simulink model "Tractor_HIT_Discrete"  (R2024a)
settings: Solver=ode1  StartTime=0.0  StopTime=60  FixedStep=0.001  RelTol=1e-3
values from neighbouring files (symbols this model uses):
  ANRtarget = 1.05    [Engine1204.sldd]    (also in Engine1204_init_r1.m; Engine2004.sldd; Engine2004_init.m; Engine3204.sldd)
  BackPrs = 3.0 4.2 5.5 7.0 8.5 10.0 11.5 12.5    [Engine1204.sldd]    (also in Engine1204_init_r1.m = [3.0, 4.2, 5.5, 7.0, 8.5, 10.0, 11.5, 12.5]; Engine2004.sldd = 3.0 4.2 5.5 7.0 8.5 10.0 11.5 12.5 13.5 14.5 15.0 15.5 16.0 ; Engine2004_init.m = [3.0,4.2,5.5,7.0,8.5,10.0,11.5,12.5,13.5,14.5,15.0,15.5,16.0; Engine3204.sldd = 3.0 4.5 6.0 7.5 9.0 10.5 12.0 13.0 13.8 14.4 14.8 15.2 15.6 )
  BackPrs_x = 50.0 100.0 150.0 200.0 250.0 300.0 350.0 400.0    [Engine1204.sldd]    (also in Engine1204_init_r1.m = [50:50:400]; Engine2004.sldd = 50.0 100.0 150.0 200.0 250.0 300.0 350.0 400.0 450.0 500.0 5; Engine2004_init.m = [50:50:800]; Engine3204.sldd = 100.0 200.0 300.0 400.0 500.0 600.0 700.0 800.0 900.0 1000.0)
  Bf = 0.38    [Engine1204.sldd]    (also in Engine2004.sldd; Engine3204.sldd)
  Br = 0.47    [Engine1204.sldd]    (also in Engine2004.sldd; Engine3204.sldd)
  BSFC = 320.0 285.0 275.0 280.0 290.0 300.0 310.0 260.0 225.0 215.0 220.0 228.0 240.0 250.0 235.0 208.0 202.0 205.0 212.0 222.0 232.0 230.0 205.0 200.0 204.0 210.0 220.0 230.0 232.0 207.0 203.0 206.0 213.0 224.0 235.0    [Engine1204.sldd]    (also in Engine1204_init_r1.m = [320,285,275,280,290,300,310; Engine2004.sldd = 315.0 280.0 270.0 275.0 285.0 295.0 305.0 255.0 220.0 210.0 ; Engine2004_init.m = [315,280,270,275,285,295,305; Engine3204.sldd = 310.0 275.0 265.0 270.0 280.0 290.0 300.0 250.0 215.0 205.0 )
  BSFC_x = 700.0 1200.0 1400.0 1600.0 1800.0 2000.0 2200.0    [Engine1204.sldd]    (also in Engine1204_init_r1.m = [700,1200,1400,1600,1800,2000,2200]; Engine2004.sldd = 800.0 1200.0 1400.0 1600.0 1800.0 2000.0 2200.0; Engine2004_init.m = [800,1200,1400,1600,1800,2000,2200]; Engine3204.sldd = 800.0 1000.0 1200.0 1400.0 1600.0 1800.0 2100.0)
  BSFC_y = 12.0 24.0 36.0 48.0 54.0    [Engine1204.sldd]    (also in Engine1204_init_r1.m = [12,24,36,48,54]; Engine2004.sldd = 20.0 40.0 60.0 80.0 100.0; Engine2004_init.m = [20,40,60,80,100]; Engine3204.sldd = 30.0 60.0 90.0 120.0 150.0)
  CO = 2.4 1.7 1.5 1.6 1.8 2.1 2.7 1.1 0.72 0.65 0.68 0.78 0.92 1.3 0.7 0.55 0.5 0.53 0.6 0.72 0.95 1.2 0.9 0.85 0.88 0.96 1.1 1.45 3.2 2.3 2.1 2.25 2.5 2.85 3.8    [Engine1204.sldd]    (also in Engine1204_init_r1.m = [; Engine2004.sldd = 2.3 1.63 1.44 1.54 1.73 2.02 2.56 1.05 0.68 0.61 0.64 0.74 0; Engine2004_init.m = [; Engine3204.sldd = 2.2 1.56 1.38 1.48 1.66 1.94 2.46 1.0 0.65 0.58 0.61 0.7 0.8)
  CO_x = 700.0 1200.0 1400.0 1600.0 1800.0 2000.0 2200.0    [Engine1204.sldd]    (also in Engine1204_init_r1.m = [700,1200,1400,1600,1800,2000,2200]; Engine2004.sldd = 800.0 1200.0 1400.0 1600.0 1800.0 2000.0 2200.0; Engine2004_init.m = [800,1200,1400,1600,1800,2000,2200]; Engine3204.sldd = 800.0 1000.0 1200.0 1400.0 1600.0 1800.0 2100.0)
  CO_y = 12.0 24.0 36.0 48.0 54.0    [Engine1204.sldd]    (also in Engine1204_init_r1.m = [12,24,36,48,54]; Engine2004.sldd = 20.0 40.0 60.0 80.0 100.0; Engine2004_init.m = [20,40,60,80,100]; Engine3204.sldd = 30.0 60.0 90.0 120.0 150.0)
  Df = 1.4    [Engine1204.sldd]    (also in Engine2004.sldd; Engine3204.sldd)
  dfmax = 0.1    [Engine1204.sldd]    (also in Engine2004.sldd; Engine3204.sldd)
  dfmin = 0.035    [Engine1204.sldd]    (also in Engine2004.sldd; Engine3204.sldd)
  DOCdPrs = 0.2 0.5 0.8 1.1 1.2    [Engine1204.sldd]    (also in Engine1204_init_r1.m = [0.2  0.5  0.8  1.1  1.2]; Engine2004.sldd = 0.25 0.55 0.85 1.15 1.3; Engine2004_init.m = [0.25,0.55,0.85,1.15,1.30]; Engine3204.sldd = 0.25 0.55 0.85 1.15 1.3 1.45)
  DOCdPrs_x = 50.0 150.0 250.0 350.0 400.0    [Engine1204.sldd]    (also in Engine1204_init_r1.m = [50  150  250  350  400]; Engine2004.sldd = 100.0 250.0 400.0 600.0 800.0; Engine2004_init.m = [100 250 400 600 800]; Engine3204.sldd = 100.0 250.0 400.0 600.0 800.0 1200.0)
  DPFdPrs = 0.3 0.5 0.7 0.9 0.6 1.0 1.4 1.8 0.9 1.5 2.1 2.6 1.2 2.0 2.7 2.8    [Engine1204.sldd]    (also in Engine1204_init_r1.m = [0.3  0.5  0.7  0.9; Engine2004.sldd = 0.35 0.6 0.85 1.1 0.7 1.15 1.6 2.0 1.05 1.7 2.3 2.5 1.4 2.2 ; Engine2004_init.m = [0.35,0.60,0.85,1.10; Engine3204.sldd = 0.35 0.7 1.05 1.4 1.7 2.0 2.2 2.4 2.55 2.65 2.7 2.75 0.6 1.1)
  DPFdPrs_x = 100.0 200.0 300.0 400.0    [Engine1204.sldd]    (also in Engine1204_init_r1.m = [100: 100 : 400]; Engine2004.sldd = 100.0 300.0 500.0 700.0; Engine2004_init.m = [100:200:700]; Engine3204.sldd = 100.0 200.0 300.0 400.0 500.0 600.0 700.0 800.0 900.0 1000.0)
  DPFdPrs_y = 0.0 6.0 12.0 20.0    [Engine1204.sldd]    (also in Engine1204_init_r1.m = [0 6 12 20 ]; Engine2004.sldd = 0.0 8.0 16.0 24.0; Engine2004_init.m = [0 8 16 24]; Engine3204.sldd = 0.0 10.0 20.0 30.0)
  DPFSootBurn = 0.0 0.0 0.0 0.0 0.0 0.2 0.4 0.6 0.8 1.0 1.2 2.4 3.6 4.8 6.0 6.0 12.0 18.0 24.0 30.0 12.0 24.0 36.0 48.0 60.0 20.0 40.0 60.0 80.0 100.0 22.0 44.0 66.0 88.0 110.0    [Engine1204.sldd]    (also in Engine1204_init_r1.m = [0,0,0,0,0; Engine2004.sldd = 0.0 0.0 0.0 0.0 0.0 0.5 1.0 1.5 2.0 2.5 3.0 6.0 9.0 12.0 15.; Engine2004_init.m = [0,0,0,0,0; Engine3204.sldd = 0.0 0.0 0.0 0.0 0.0 0.5 1.0 1.5 2.0 2.5 3.0 6.0 9.0 12.0 15.)
  DPFSootBurn_x = 100.0 200.0 300.0 400.0 500.0    [Engine1204.sldd]    (also in Engine1204_init_r1.m = [100,200,300,400,500]; Engine2004.sldd = 200.0 300.0 400.0 500.0 650.0; Engine2004_init.m = [200,300,400,500,650]; Engine3204.sldd = 200.0 300.0 400.0 500.0 650.0)
  DPFSootBurn_y = 400.0 450.0 500.0 550.0 600.0 650.0 680.0    [Engine1204.sldd]    (also in Engine1204_init_r1.m = [400,450,500,550,600,650,680]; Engine2004.sldd; Engine2004_init.m = [400,450,500,550,600,650,680]; Engine3204.sldd)
  Dr = 1.8    [Engine1204.sldd]    (also in Engine2004.sldd; Engine3204.sldd)
  drmax = 0.12    [Engine1204.sldd]    (also in Engine2004.sldd; Engine3204.sldd)
  drmin = 0.04    [Engine1204.sldd]    (also in Engine2004.sldd; Engine3204.sldd)
  EGRKi = 0.03    [Engine1204.sldd]    (also in Engine1204_init_r1.m; Engine2004.sldd; Engine2004_init.m; Engine3204.sldd)
  EGRKp = 3.5999999999999996    [Engine1204.sldd]    (also in Engine1204_init_r1.m = 3.6; Engine2004.sldd; Engine2004_init.m = 3.6; Engine3204.sldd)
  EGRMax = 1.0    [Engine1204.sldd]    (also in Engine1204_init_r1.m = 1; Engine2004.sldd; Engine2004_init.m = 1; Engine3204.sldd)
  EGRMin = 0.0    [Engine1204.sldd]    (also in Engine1204_init_r1.m = 0; Engine2004.sldd; Engine2004_init.m = 0; Engine3204.sldd)
  EGRRatio = 0.0 0.0 0.0 0.0 0.0 0.0 0.0 0.0 0.04 0.03 0.03 0.02 0.02 0.01 0.0 0.08 0.07 0.06 0.05 0.04 0.03 0.0 0.13 0.12 0.11 0.1 0.09 0.08 0.0 0.18 0.17 0.16 0.15 0.14 0.13 0.0 0.22 0.21 0.2 0.19 0.18 0.17    [Engine1204.sldd]    (also in Engine1204_init_r1.m = [; Engine2004.sldd; Engine2004_init.m = [; Engine3204.sldd)
  EGRRatio_x = 700.0 1200.0 1400.0 1600.0 1800.0 2000.0 2200.0    [Engine1204.sldd]    (also in Engine1204_init_r1.m = [700,1200,1400,1600,1800,2000,2200]; Engine2004.sldd = 800.0 1200.0 1400.0 1600.0 1800.0 2000.0 2200.0; Engine2004_init.m = [800,1200,1400,1600,1800,2000,2200]; Engine3204.sldd = 800.0 1000.0 1200.0 1400.0 1600.0 1800.0 2100.0)
  EGRRatio_y = 0.0 20.0 40.0 60.0 80.0 100.0    [Engine1204.sldd]    (also in Engine1204_init_r1.m = [0,20,40,60,80,100]; Engine2004.sldd; Engine2004_init.m = [0,20,40,60,80,100]; Engine3204.sldd)
  EGRTgt = 0.25 0.22 0.2 0.18 0.16 0.12 0.1 0.2 0.18 0.15 0.14 0.12 0.1 0.08 0.12 0.13 0.1 0.09 0.08 0.06 0.04 0.08 0.09 0.07 0.06 0.05 0.03 0.02 0.05 0.06 0.04 0.03 0.02 0.01 0.0    [Engine1204.sldd]    (also in Engine1204_init_r1.m = [0.25,0.22,0.20,0.18,0.16,0.12,0.10; Engine2004.sldd = 0.24 0.21 0.19 0.17 0.15 0.11 0.09 0.19 0.17 0.14 0.13 0.11 ; Engine2004_init.m = [0.24,0.21,0.19,0.17,0.15,0.11,0.09; Engine3204.sldd = 0.23 0.2 0.18 0.16 0.14 0.1 0.08 0.18 0.16 0.13 0.12 0.1 0.0)
  EGRTgt_x = 700.0 1200.0 1400.0 1600.0 1800.0 2000.0 2200.0    [Engine1204.sldd]    (also in Engine1204_init_r1.m = [700,1200,1400,1600,1800,2000,2200]; Engine2004.sldd = 800.0 1200.0 1400.0 1600.0 1800.0 2000.0 2200.0; Engine2004_init.m = [800,1200,1400,1600,1800,2000,2200]; Engine3204.sldd = 800.0 1000.0 1200.0 1400.0 1600.0 1800.0 2100.0)
  EGRTgt_y = 12.0 24.0 36.0 48.0 54.0    [Engine1204.sldd]    (also in Engine1204_init_r1.m = [12,24,36,48,54]; Engine2004.sldd = 20.0 40.0 60.0 80.0 100.0; Engine2004_init.m = [20,40,60,80,100]; Engine3204.sldd = 30.0 60.0 90.0 120.0 150.0)
  EGT = 197.0 257.0 287.0 297.0 287.0 267.0 247.0 267.0 357.0 397.0 407.0 392.0 367.0 347.0 337.0 437.0 472.0 482.0 462.0 437.0 407.0 367.0 477.0 502.0 512.0 492.0 467.0 437.0 377.0 487.0 510.0 520.0 500.0 477.0 447.0    [Engine1204.sldd]    (also in Engine1204_init_r1.m = [470,530,560,570,560,540,520; Engine2004.sldd = 187.0 247.0 277.0 287.0 277.0 257.0 237.0 257.0 347.0 387.0 ; Engine2004_init.m = [460,520,550,560,550,530,510; Engine3204.sldd = 307.0 327.0 338.0 327.0 307.0 277.0 237.0 322.0 337.0 332.0 )
  EGT_x = 700.0 1200.0 1400.0 1600.0 1800.0 2000.0 2200.0    [Engine1204.sldd]    (also in Engine1204_init_r1.m = [700,1200,1400,1600,1800,2000,2200]; Engine2004.sldd = 800.0 1200.0 1400.0 1600.0 1800.0 2000.0 2200.0; Engine2004_init.m = [800,1200,1400,1600,1800,2000,2200]; Engine3204.sldd = 800.0 1000.0 1200.0 1400.0 1600.0 1800.0 2100.0)
  EGT_y = 12.0 24.0 36.0 48.0 54.0    [Engine1204.sldd]    (also in Engine1204_init_r1.m = [12,24,36,48,54]; Engine2004.sldd = 20.0 40.0 60.0 80.0 100.0; Engine2004_init.m = [20,40,60,80,100]; Engine3204.sldd = 30.0 60.0 90.0 120.0 150.0)
  EngCsup = 0.35594 0.35501499999999997 0.353535 0.35242500000000004 0.351685 0.35150000000000003 0.35187 0.352795 0.35446 0.356865    [Engine1204.sldd]    (also in Engine2004.sldd; Engine3204.sldd)
  EngineSpdTgt = 700.0 850.0 1000.0 1150.0 1300.0 1450.0 1600.0 1750.0 1900.0 2050.0 2200.0    [Engine1204.sldd]    (also in Engine1204_init_r1.m = [700:150:2200]; Engine2004.sldd; Engine2004_init.m = [700:150:2200]; Engine3204.sldd = 800.0 930.0 1060.0 1190.0 1320.0 1450.0 1580.0 1710.0 1840.0)
  EngineSpdTgt_x = 0.0 10.0 20.0 30.0 40.0 50.0 60.0 70.0 80.0 90.0 100.0    [Engine1204.sldd]    (also in Engine1204_init_r1.m = [0:10:100]; Engine2004.sldd; Engine2004_init.m = [0:10:100]; Engine3204.sldd)
  EngineTrq = 70.0 110.0 130.0 125.0 115.0 100.0 85.0 180.0 280.0 320.0 310.0 285.0 250.0 220.0 260.0 370.0 410.0 395.0 365.0 320.0 280.0 300.0 420.0 450.0 435.0 400.0 350.0 300.0 310.0 435.0 460.0 445.0 410.0 355.0 305.0    [Engine1204.sldd]    (also in Engine1204_init_r1.m = [70,110,130,125,115,100,85; Engine2004.sldd = 130.0 200.0 240.0 230.0 210.0 180.0 150.0 320.0 480.0 550.0 ; Engine2004_init.m = [130,200,240,230,210,180,150; Engine3204.sldd = 210.0 320.0 380.0 360.0 330.0 290.0 240.0 510.0 760.0 870.0 )
  EngineTrq_x = 700.0 1200.0 1400.0 1600.0 1800.0 2000.0 2200.0    [Engine1204.sldd]    (also in Engine1204_init_r1.m = [700,1200,1400,1600,1800,2000,2200]; Engine2004.sldd = 800.0 1200.0 1400.0 1600.0 1800.0 2000.0 2200.0; Engine2004_init.m = [800,1200,1400,1600,1800,2000,2200]; Engine3204.sldd = 800.0 1000.0 1200.0 1400.0 1600.0 1800.0 2100.0)
  EngineTrq_y = 12.0 24.0 36.0 48.0 54.0    [Engine1204.sldd]    (also in Engine1204_init_r1.m = [12,24,36,48,54]; Engine2004.sldd = 20.0 40.0 60.0 80.0 100.0; Engine2004_init.m = [20,40,60,80,100]; Engine3204.sldd = 30.0 60.0 90.0 120.0 150.0)
  EngSpd = 800.0 1000.0 1200.0 1400.0 1600.0 1800.0 2000.0 2200.0 2400.0 2600.0    [Engine1204.sldd]    (also in Engine2004.sldd; Engine3204.sldd)
  EngTrq = 667.0 700.0 768.0 830.0 885.0 860.0 789.0 690.0 542.0 352.0    [Engine1204.sldd]    (also in Engine2004.sldd; Engine3204.sldd)
  etaCO = 0.0 0.0 0.0 0.0 0.6 0.45 0.3 0.15 0.92 0.85 0.75 0.6 0.98 0.95 0.9 0.82 0.99 0.97 0.94 0.88    [Engine1204.sldd]    (also in Engine1204_init_r1.m = [0.00	0.00	0.00	0.00; Engine2004.sldd; Engine2004_init.m = [0.00	0.00	0.00	0.00; Engine3204.sldd)
  etaCO_x = 10000.0 25000.0 40000.0 60000.0    [Engine1204.sldd]    (also in Engine1204_init_r1.m = [10000  25000  40000  60000]; Engine2004.sldd; Engine2004_init.m = [10000 25000 40000 60000]; Engine3204.sldd)
  etaCO_y = 120.0 200.0 280.0 360.0 450.0    [Engine1204.sldd]    (also in Engine1204_init_r1.m = [120, 200, 280, 360, 450]; Engine2004.sldd; Engine2004_init.m = [120,200,280,360,450]; Engine3204.sldd)
  etaHC = 0.0 0.0 0.0 0.0 0.5 0.35 0.2 0.1 0.88 0.8 0.68 0.5 0.96 0.92 0.86 0.75 0.98 0.95 0.91 0.83    [Engine1204.sldd]    (also in Engine1204_init_r1.m = [0.00	0.00	0.00	0.00; Engine2004.sldd; Engine2004_init.m = [0.00	0.00	0.00	0.00; Engine3204.sldd)
  etaHC_x = 10000.0 25000.0 40000.0 60000.0    [Engine1204.sldd]    (also in Engine1204_init_r1.m = [10000  25000  40000  60000]; Engine2004.sldd; Engine2004_init.m = [10000 25000 40000 60000]; Engine3204.sldd)
  etaHC_y = 120.0 200.0 280.0 360.0 450.0    [Engine1204.sldd]    (also in Engine1204_init_r1.m = [120, 200, 280, 360, 450]; Engine2004.sldd; Engine2004_init.m = [120,200,280,360,450]; Engine3204.sldd)
  etaNO2 = 0.0 0.0 0.0 0.0 0.2 0.15 0.1 0.05 0.4 0.33 0.25 0.18 0.55 0.48 0.4 0.3 0.6 0.53 0.45 0.35    [Engine1204.sldd]    (also in Engine1204_init_r1.m = [0.00	0.00	0.00	0.00; Engine2004.sldd; Engine2004_init.m = [0.00	0.00	0.00	0.00; Engine3204.sldd)
  etaNO2_x = 10000.0 25000.0 40000.0 60000.0    [Engine1204.sldd]    (also in Engine1204_init_r1.m = [10000  25000  40000  60000]; Engine2004.sldd; Engine2004_init.m = [10000 25000 40000 60000]; Engine3204.sldd)
  etaNO2_y = 120.0 200.0 280.0 360.0 450.0    [Engine1204.sldd]    (also in Engine1204_init_r1.m = [120, 200, 280, 360, 450]; Engine2004.sldd; Engine2004_init.m = [120,200,280,360,450]; Engine3204.sldd)
  etaPM = 0.995 0.992 0.988 0.98 0.996 0.994 0.99 0.985 0.997 0.995 0.992 0.988    [Engine1204.sldd]    (also in Engine1204_init_r1.m = [0.995  0.992  0.988  0.980; Engine2004.sldd; Engine2004_init.m = [0.995  0.992  0.988  0.980; Engine3204.sldd)
  etaPM_x = 10000.0 25000.0 40000.0 60000.0    [Engine1204.sldd]    (also in Engine1204_init_r1.m = [10000  25000  40000  60000]; Engine2004.sldd; Engine2004_init.m = [10000 25000 40000 60000]; Engine3204.sldd)
  etaPM_y = 150.0 300.0 450.0    [Engine1204.sldd]    (also in Engine1204_init_r1.m = [150, 300, 450]; Engine2004.sldd; Engine2004_init.m = [150,300,450]; Engine3204.sldd)
  FuelCyleMax = 40.0 45.0 50.0 52.0 54.0 50.0 60.0 65.0 66.0 68.0 52.0 64.0 66.0 67.0 68.0 50.0 62.0 64.0 65.0 66.0 48.0 58.0 60.0 61.0 62.0 42.0 50.0 52.0 53.0 54.0 38.0 44.0 46.0 47.0 48.0    [Engine1204.sldd]    (also in Engine1204_init_r1.m = [40,45,50,52,54; Engine2004.sldd = 65.0 75.0 82.0 88.0 92.0 75.0 88.0 94.0 98.0 102.0 78.0 92.0; Engine2004_init.m = [65,75,82,88,92; Engine3204.sldd = 95.0 110.0 125.0 140.0 155.0 110.0 130.0 145.0 160.0 175.0 1)
  FuelCyleMax_x = 80.0 140.0 200.0 260.0 320.0    [Engine1204.sldd]    (also in Engine1204_init_r1.m = [80,140,200,260,320]; Engine2004.sldd = 150.0 300.0 450.0 600.0 750.0; Engine2004_init.m = [150,300,450,600,750]; Engine3204.sldd = 250.0 500.0 750.0 1000.0 1300.0)
  FuelCyleMax_y = 700.0 1200.0 1400.0 1600.0 1800.0 2000.0 2200.0    [Engine1204.sldd]    (also in Engine1204_init_r1.m = [700,1200,1400,1600,1800,2000,2200]; Engine2004.sldd = 800.0 1200.0 1400.0 1600.0 1800.0 2000.0 2200.0; Engine2004_init.m = [800,1200,1400,1600,1800,2000,2200]; Engine3204.sldd = 800.0 1000.0 1200.0 1400.0 1600.0 1800.0 2100.0)
  FuelCyleMaxSw = 0.0    [Engine1204.sldd]    (also in Engine1204_init_r1.m = 0; Engine2004.sldd; Engine2004_init.m = 0; Engine3204.sldd)
  FuelCyleMin = 10.0    [Engine1204.sldd]    (also in Engine1204_init_r1.m = 10; Engine2004.sldd = 12.0; Engine2004_init.m = 12; Engine3204.sldd = 15.0)
  FuelKd = 0.0    [Engine1204.sldd]    (also in Engine1204_init_r1.m = 0; Engine2004.sldd; Engine2004_init.m = 0; Engine3204.sldd)
  FuelKi = 0.0162    [Engine1204.sldd]    (also in Engine1204_init_r1.m; Engine2004.sldd = 0.0198; Engine2004_init.m = 0.0198; Engine3204.sldd = 0.025199999999999997)
  FuelKp = 0.054    [Engine1204.sldd]    (also in Engine1204_init_r1.m; Engine2004.sldd = 0.066; Engine2004_init.m = 0.066; Engine3204.sldd = 0.083999999999999991)
  g = 9.81    [Engine1204.sldd]    (also in Engine2004.sldd; Engine3204.sldd)
  GearA = -2.9 0.0 6.0 2.5 1.0    [Engine1204.sldd]    (also in Engine2004.sldd; Engine3204.sldd)
  GearAC = -1.0 0.0 1.0 2.0 3.0    [Engine1204.sldd]    (also in Engine2004.sldd; Engine3204.sldd)
  GearFront = 17.574    [Engine1204.sldd]    (also in Engine2004.sldd; Engine3204.sldd)
  GearM = 2.33 1.75 1.4 1.0    [Engine1204.sldd]    (also in Engine2004.sldd; Engine3204.sldd)
  GearMC = 1.0 2.0 3.0 4.0    [Engine1204.sldd]    (also in Engine2004.sldd; Engine3204.sldd)
  GearRef = 14.6    [Engine1204.sldd]    (also in Engine2004.sldd; Engine3204.sldd)
  HC = 0.85 0.6 0.52 0.55 0.62 0.7 0.9 0.4 0.22 0.2 0.21 0.26 0.32 0.48 0.25 0.18 0.17 0.18 0.21 0.26 0.36 0.32 0.24 0.23 0.25 0.28 0.33 0.42 0.55 0.42 0.4 0.43 0.48 0.54 0.68    [Engine1204.sldd]    (also in Engine1204_init_r1.m = [; Engine2004.sldd = 0.82 0.58 0.5 0.53 0.6 0.68 0.87 0.38 0.21 0.19 0.2 0.24 0.3; Engine2004_init.m = [; Engine3204.sldd = 0.8 0.56 0.48 0.51 0.58 0.66 0.84 0.37 0.2 0.18 0.19 0.23 0.)
  HC_x = 700.0 1200.0 1400.0 1600.0 1800.0 2000.0 2200.0    [Engine1204.sldd]    (also in Engine1204_init_r1.m = [700,1200,1400,1600,1800,2000,2200]; Engine2004.sldd = 800.0 1200.0 1400.0 1600.0 1800.0 2000.0 2200.0; Engine2004_init.m = [800,1200,1400,1600,1800,2000,2200]; Engine3204.sldd = 800.0 1000.0 1200.0 1400.0 1600.0 1800.0 2100.0)
  HC_y = 12.0 24.0 36.0 48.0 54.0    [Engine1204.sldd]    (also in Engine1204_init_r1.m = [12,24,36,48,54]; Engine2004.sldd = 20.0 40.0 60.0 80.0 100.0; Engine2004_init.m = [20,40,60,80,100]; Engine3204.sldd = 30.0 60.0 90.0 120.0 150.0)
  hf = 0.35    [Engine1204.sldd]    (also in Engine2004.sldd; Engine3204.sldd)
  hr = 0.4    [Engine1204.sldd]    (also in Engine2004.sldd; Engine3204.sldd)
  IdleEngSpd = 700.0    [Engine1204.sldd]    (also in Engine2004.sldd; Engine3204.sldd)
  IdleThrottle = 0.3    [Engine1204.sldd]    (also in Engine2004.sldd; Engine3204.sldd)
  Inertia = 0.9    [Engine1204.sldd]    (also in Engine1204_init_r1.m; Engine2004.sldd = 1.4; Engine2004_init.m = 1.4; Engine3204.sldd = 2.0)
  Intake = 80.0 140.0 160.0 180.0 190.0 195.0 200.0 130.0 210.0 240.0 260.0 270.0 275.0 280.0 170.0 270.0 310.0 330.0 340.0 345.0 350.0 190.0 320.0 360.0 380.0 390.0 395.0 400.0 200.0 340.0 380.0 400.0 410.0 415.0 420.0    [Engine1204.sldd]    (also in Engine1204_init_r1.m = [80,140,160,180,190,195,200; Engine2004.sldd = 160.0 240.0 280.0 310.0 330.0 340.0 350.0 250.0 380.0 440.0 ; Engine2004_init.m = [160,240,280,310,330,340,350; Engine3204.sldd = 280.0 420.0 490.0 540.0 570.0 585.0 600.0 430.0 660.0 760.0 )
  Intake_x = 700.0 1200.0 1400.0 1600.0 1800.0 2000.0 2200.0    [Engine1204.sldd]    (also in Engine1204_init_r1.m = [700,1200,1400,1600,1800,2000,2200]; Engine2004.sldd = 800.0 1200.0 1400.0 1600.0 1800.0 2000.0 2200.0; Engine2004_init.m = [800,1200,1400,1600,1800,2000,2200]; Engine3204.sldd = 800.0 1000.0 1200.0 1400.0 1600.0 1800.0 2100.0)
  Intake_y = 12.0 24.0 36.0 48.0 54.0    [Engine1204.sldd]    (also in Engine1204_init_r1.m = [12,24,36,48,54]; Engine2004.sldd = 20.0 40.0 60.0 80.0 100.0; Engine2004_init.m = [20,40,60,80,100]; Engine3204.sldd = 30.0 60.0 90.0 120.0 150.0)
  IntakePrs = 1.0 1.1 1.22 1.35 1.48 1.6 1.7 1.0 1.12 1.24 1.37 1.5 1.62 1.72 1.0 1.13 1.25 1.38 1.51 1.63 1.73 1.0 1.14 1.26 1.39 1.52 1.64 1.74 1.0 1.15 1.27 1.4 1.53 1.65 1.75 1.0 1.16 1.28 1.41 1.54 1.66 1.76    [Engine1204.sldd]    (also in Engine1204_init_r1.m = [; Engine2004.sldd = 1.0 1.11 1.23 1.36 1.49 1.61 1.71 1.0 1.13 1.25 1.38 1.51 1.; Engine2004_init.m = [; Engine3204.sldd = 1.0 1.12 1.24 1.37 1.5 1.62 1.72 1.0 1.14 1.26 1.39 1.52 1.6)
  IntakePrs_x = 700.0 1200.0 1400.0 1600.0 1800.0 2000.0 2200.0    [Engine1204.sldd]    (also in Engine1204_init_r1.m = [700,1200,1400,1600,1800,2000,2200]; Engine2004.sldd = 800.0 1200.0 1400.0 1600.0 1800.0 2000.0 2200.0; Engine2004_init.m = [800,1200,1400,1600,1800,2000,2200]; Engine3204.sldd = 800.0 1000.0 1200.0 1400.0 1600.0 1800.0 2100.0)
  IntakePrs_y = 0.0 20.0 40.0 60.0 80.0 100.0    [Engine1204.sldd]    (also in Engine1204_init_r1.m = [0,20,40,60,80,100]; Engine2004.sldd; Engine2004_init.m = [0,20,40,60,80,100]; Engine3204.sldd)
  IntakePrsInit = 1.35    [Engine1204.sldd]    (also in Engine1204_init_r1.m; Engine2004.sldd; Engine2004_init.m; Engine3204.sldd)
  IntakeSw = 0    [Engine1204.sldd]    (also in Engine1204_init_r1.m = false; Engine2004.sldd; Engine2004_init.m = false; Engine3204.sldd)
  IntakeTC = 0.1    [Engine1204.sldd]    (also in Engine1204_init_r1.m; Engine2004.sldd; Engine2004_init.m; Engine3204.sldd)
  IntakeTemp = 25.0 28.0 30.0 32.0 34.0 36.0 38.0 25.0 38.0 40.0 42.0 44.0 46.0 48.0 25.0 48.0 50.0 52.0 54.0 56.0 58.0 25.0 58.0 60.0 62.0 64.0 66.0 68.0 25.0 66.0 68.0 70.0 72.0 74.0 76.0 25.0 72.0 74.0 76.0 78.0 80.0 82.0    [Engine1204.sldd]    (also in Engine1204_init_r1.m = [; Engine2004.sldd = 25.0 29.0 31.0 33.0 35.0 37.0 39.0 25.0 39.0 41.0 43.0 45.0 ; Engine2004_init.m = [; Engine3204.sldd = 25.0 30.0 32.0 34.0 36.0 38.0 40.0 25.0 40.0 42.0 44.0 46.0 )
  IntakeTemp_x = 700.0 1200.0 1400.0 1600.0 1800.0 2000.0 2200.0    [Engine1204.sldd]    (also in Engine1204_init_r1.m = [700,1200,1400,1600,1800,2000,2200]; Engine2004.sldd = 800.0 1200.0 1400.0 1600.0 1800.0 2000.0 2200.0; Engine2004_init.m = [800,1200,1400,1600,1800,2000,2200]; Engine3204.sldd = 800.0 1000.0 1200.0 1400.0 1600.0 1800.0 2100.0)
  IntakeTemp_y = 0.0 20.0 40.0 60.0 80.0 100.0    [Engine1204.sldd]    (also in Engine1204_init_r1.m = [0,20,40,60,80,100]; Engine2004.sldd; Engine2004_init.m = [0,20,40,60,80,100]; Engine3204.sldd)
  IntakeTempInit = 45.0    [Engine1204.sldd]    (also in Engine1204_init_r1.m = 45; Engine2004.sldd; Engine2004_init.m = 45; Engine3204.sldd)
  Jf = 180.0    [Engine1204.sldd]    (also in Engine2004.sldd; Engine3204.sldd)
  Jr = 450.0    [Engine1204.sldd]    (also in Engine2004.sldd; Engine3204.sldd)
  L = 2.75    [Engine1204.sldd]    (also in Engine2004.sldd; Engine3204.sldd)
  LiftTorque = 5000.0    [Engine1204.sldd]    (also in Engine2004.sldd; Engine3204.sldd)
  LoadTrqManu = 200.0    [Engine1204.sldd]    (also in Engine1204_init_r1.m = 200; Engine2004.sldd = 400.0; Engine2004_init.m = 400; Engine3204.sldd = 800.0)
  LoadTrqSW = 1    [Engine1204.sldd]    (also in Engine1204_init_r1.m = true; Engine2004.sldd; Engine2004_init.m = true; Engine3204.sldd = 0)
  M_I = 2500.0    [Engine1204.sldd]    (also in Engine2004.sldd; Engine3204.sldd)
  M_T = 6500.0    [Engine1204.sldd]    (also in Engine2004.sldd; Engine3204.sldd)
  MaxEngSpd = 2600.0    [Engine1204.sldd]    (also in Engine2004.sldd; Engine3204.sldd)
  NH3StoreMax = 0.0 1.2 2.0 2.4 2.2 1.7 1.1    [Engine1204.sldd]    (also in Engine1204_init_r1.m = [0  1.2  2.0  2.4  2.2  1.7  1.1]; Engine2004.sldd = 0.0 1.7 2.9 3.5 3.2 2.5 1.6; Engine2004_init.m = [0, 1.7, 2.9, 3.5, 3.2, 2.5, 1.6]; Engine3204.sldd = 0.0 2.2 3.8 4.5 4.2 3.3 2.1)
  NH3StoreMax_x = 180.0 220.0 260.0 300.0 340.0 380.0 420.0    [Engine1204.sldd]    (also in Engine1204_init_r1.m = [180  220  260  300  340  380  420]; Engine2004.sldd; Engine2004_init.m = [180 220 260 300 340 380 420]; Engine3204.sldd)
  NOx = 6.2 7.0 7.4 7.2 6.8 6.4 6.0 7.5 8.4 8.8 8.6 8.2 7.7 7.2 8.2 9.1 9.5 9.3 8.9 8.4 7.9 7.6 8.5 8.8 8.6 8.2 7.7 7.2 7.0 7.8 8.1 7.9 7.5 7.0 6.5    [Engine1204.sldd]    (also in Engine1204_init_r1.m = [6.2,7.0,7.4,7.2,6.8,6.4,6.0; Engine2004.sldd = 6.1 6.9 7.3 7.1 6.7 6.3 5.9 7.4 8.3 8.7 8.5 8.1 7.6 7.1 8.1 ; Engine2004_init.m = [6.1,6.9,7.3,7.1,6.7,6.3,5.9; Engine3204.sldd = 5.9 6.7 7.1 6.9 6.5 6.1 5.7 7.2 8.1 8.5 8.3 7.9 7.4 6.9 7.9 )
  NOx_x = 700.0 1200.0 1400.0 1600.0 1800.0 2000.0 2200.0    [Engine1204.sldd]    (also in Engine1204_init_r1.m = [700,1200,1400,1600,1800,2000,2200]; Engine2004.sldd = 800.0 1200.0 1400.0 1600.0 1800.0 2000.0 2200.0; Engine2004_init.m = [800,1200,1400,1600,1800,2000,2200]; Engine3204.sldd = 800.0 1000.0 1200.0 1400.0 1600.0 1800.0 2100.0)
  NOx_y = 12.0 24.0 36.0 48.0 54.0    [Engine1204.sldd]    (also in Engine1204_init_r1.m = [12,24,36,48,54]; Engine2004.sldd = 20.0 40.0 60.0 80.0 100.0; Engine2004_init.m = [20,40,60,80,100]; Engine3204.sldd = 30.0 60.0 90.0 120.0 150.0)
  NOxFac = 1.0 0.88 0.76 0.64 0.54 0.46 0.4    [Engine1204.sldd]    (also in Engine1204_init_r1.m = [1.00, 0.88, 0.76, 0.64, 0.54, 0.46, 0.40]; Engine2004.sldd; Engine2004_init.m = [1.00,0.88,0.76,0.64,0.54,0.46,0.40]; Engine3204.sldd)
  NOxFac_x = 0.0 0.05 0.1 0.15 0.19999999999999998 0.25 0.3    [Engine1204.sldd]    (also in Engine1204_init_r1.m = [0: 0.05 : 0.3]; Engine2004.sldd; Engine2004_init.m = [0:0.05:0.3]; Engine3204.sldd)
  NumCyl = 6.0    [Engine1204.sldd]    (also in Engine1204_init_r1.m = 6; Engine2004.sldd; Engine2004_init.m = 6; Engine3204.sldd)
  O2 = 16.5 16.0 15.8 15.5 15.2 14.8 14.5 13.0 12.2 11.8 11.5 11.2 10.8 10.5 9.5 8.6 8.0 7.7 7.4 7.0 6.7 7.0 6.2 5.6 5.3 5.0 4.7 4.4 6.0 5.3 4.8 4.5 4.2 4.0 3.8    [Engine1204.sldd]    (also in Engine1204_init_r1.m = [16.5,16.0,15.8,15.5,15.2,14.8,14.5; Engine2004.sldd = 16.3 15.8 15.6 15.3 15.0 14.6 14.3 12.8 12.0 11.6 11.3 11.0 ; Engine2004_init.m = [16.3,15.8,15.6,15.3,15.0,14.6,14.3; Engine3204.sldd = 16.0 15.5 15.3 15.0 14.7 14.3 14.0 12.5 11.7 11.3 11.0 10.7 )
  O2_x = 700.0 1200.0 1400.0 1600.0 1800.0 2000.0 2200.0    [Engine1204.sldd]    (also in Engine1204_init_r1.m = [700,1200,1400,1600,1800,2000,2200]; Engine2004.sldd = 800.0 1200.0 1400.0 1600.0 1800.0 2000.0 2200.0; Engine2004_init.m = [800,1200,1400,1600,1800,2000,2200]; Engine3204.sldd = 800.0 1000.0 1200.0 1400.0 1600.0 1800.0 2100.0)
  O2_y = 12.0 24.0 36.0 48.0 54.0    [Engine1204.sldd]    (also in Engine1204_init_r1.m = [12,24,36,48,54]; Engine2004.sldd = 20.0 40.0 60.0 80.0 100.0; Engine2004_init.m = [20,40,60,80,100]; Engine3204.sldd = 30.0 60.0 90.0 120.0 150.0)
  PM = 0.12 0.1 0.09 0.09 0.1 0.11 0.12 0.22 0.18 0.16 0.17 0.19 0.21 0.24 0.38 0.3 0.26 0.27 0.31 0.35 0.39 0.55 0.44 0.38 0.4 0.45 0.5 0.56 0.65 0.52 0.46 0.48 0.53 0.58 0.66    [Engine1204.sldd]    (also in Engine1204_init_r1.m = [0.12,0.10,0.09,0.09,0.10,0.11,0.12; Engine2004.sldd = 0.11 0.09 0.08 0.08 0.09 0.1 0.11 0.21 0.17 0.15 0.16 0.18 0; Engine2004_init.m = [0.11,0.09,0.08,0.08,0.09,0.10,0.11; Engine3204.sldd = 0.1 0.08 0.07 0.07 0.08 0.09 0.1 0.2 0.16 0.14 0.15 0.17 0.1)
  PM_x = 700.0 1200.0 1400.0 1600.0 1800.0 2000.0 2200.0    [Engine1204.sldd]    (also in Engine1204_init_r1.m = [700,1200,1400,1600,1800,2000,2200]; Engine2004.sldd = 800.0 1200.0 1400.0 1600.0 1800.0 2000.0 2200.0; Engine2004_init.m = [800,1200,1400,1600,1800,2000,2200]; Engine3204.sldd = 800.0 1000.0 1200.0 1400.0 1600.0 1800.0 2100.0)
  PM_y = 12.0 24.0 36.0 48.0 54.0    [Engine1204.sldd]    (also in Engine1204_init_r1.m = [12,24,36,48,54]; Engine2004.sldd = 20.0 40.0 60.0 80.0 100.0; Engine2004_init.m = [20,40,60,80,100]; Engine3204.sldd = 30.0 60.0 90.0 120.0 150.0)
  radps2rpm = 9.55    [Engine1204.sldd]    (also in Engine1204_init_r1.m; Engine2004.sldd; Engine2004_init.m; Engine3204.sldd)
  RailFuel = 400.0 600.0 700.0 700.0 650.0 600.0 550.0 600.0 800.0 900.0 900.0 850.0 800.0 750.0 700.0 1000.0 1100.0 1150.0 1100.0 1000.0 950.0 750.0 1200.0 1350.0 1350.0 1300.0 1200.0 1150.0 750.0 1300.0 1400.0 1450.0 1400.0 1300.0 1200.0    [Engine1204.sldd]    (also in Engine1204_init_r1.m = [400,600,700,700,650,600,550; Engine2004.sldd = 420.0 620.0 720.0 720.0 680.0 630.0 580.0 630.0 830.0 930.0 ; Engine2004_init.m = [420,620,720,720,680,630,580; Engine3204.sldd = 440.0 640.0 740.0 740.0 700.0 650.0 600.0 650.0 850.0 950.0 )
  RailFuel_x = 700.0 1200.0 1400.0 1600.0 1800.0 2000.0 2200.0    [Engine1204.sldd]    (also in Engine1204_init_r1.m = [700,1200,1400,1600,1800,2000,2200]; Engine2004.sldd = 800.0 1200.0 1400.0 1600.0 1800.0 2000.0 2200.0; Engine2004_init.m = [800,1200,1400,1600,1800,2000,2200]; Engine3204.sldd = 800.0 1000.0 1200.0 1400.0 1600.0 1800.0 2100.0)
  ... (+23 more)
undefined symbols (not defined in the file or in its folder): df, DiscIntNeverNeededParam, dr, MAP_AIR, MAP_EFF, MAP_EoCO, MAP_EoCO2, MAP_EoHC, MAP_EoNOx, MAP_EoPM, MAP_FUEL, MAP_FUELCMD, MAP_POWER, MAP_SPD, MAP_TEMPERATURE, NH3_MAX, R
libraries: simulink x9, slpidlib x5
(part 2 of 10)

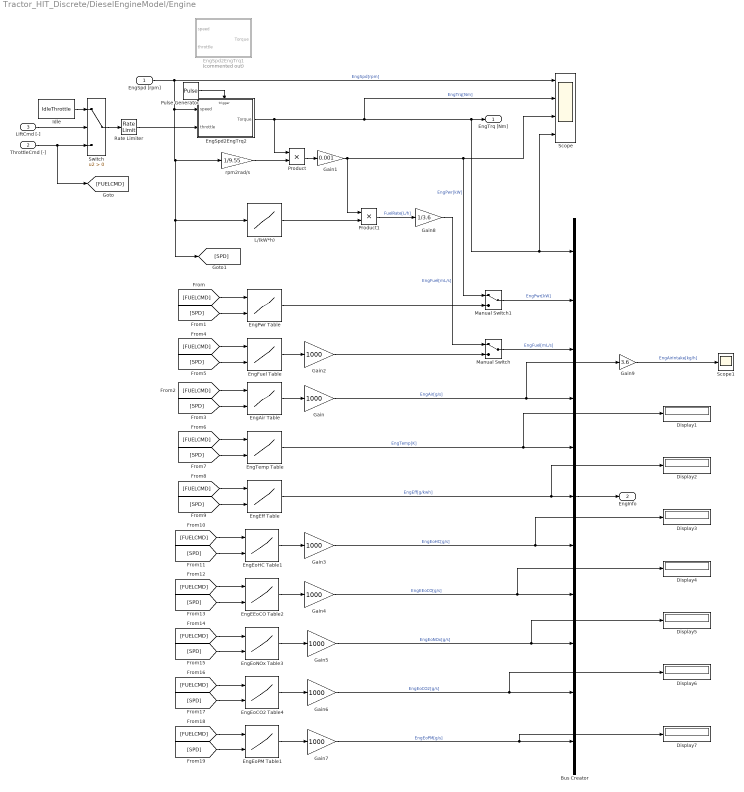
== system Tractor_HIT_Discrete/DieselEngineModel/Engine ==
  EngSpd [rpm] : Inport
  ThrottleCmd [-] : Inport  Port=2
  LiftCmd [-] : Inport  Port=3
  Bus Creator : BusCreator  Inputs=11
  Display{1..7} (7 alike) : Display
  EngAir Table : Lookup_n-D  BreakpointsForDimension1=MAP_FUELCMD  BreakpointsForDimension2=MAP_SPD  Table=MAP_AIR  ExtrapMethod=Clip  InternalRulePriority=Speed  RndMeth=Simplest
      settings: InputPortMap=u0,u1
  EngEEoCO Table2 : Lookup_n-D  BreakpointsForDimension1=MAP_FUELCMD  BreakpointsForDimension2=MAP_SPD  Table=MAP_EoCO  ExtrapMethod=Clip  InternalRulePriority=Speed  RndMeth=Simplest
      settings: InputPortMap=u0,u1
  EngEff Table : Lookup_n-D  BreakpointsForDimension1=MAP_FUELCMD  BreakpointsForDimension2=MAP_SPD  Table=MAP_EFF  ExtrapMethod=Clip  InternalRulePriority=Speed  RndMeth=Simplest
      settings: InputPortMap=u0,u1
  EngEoCO2 Table4 : Lookup_n-D  BreakpointsForDimension1=MAP_FUELCMD  BreakpointsForDimension2=MAP_SPD  Table=MAP_EoCO2  ExtrapMethod=Clip  InternalRulePriority=Speed  RndMeth=Simplest
      settings: InputPortMap=u0,u1
  EngEoHC Table1 : Lookup_n-D  BreakpointsForDimension1=MAP_FUELCMD  BreakpointsForDimension2=MAP_SPD  Table=MAP_EoHC  ExtrapMethod=Clip  InternalRulePriority=Speed  RndMeth=Simplest
      settings: InputPortMap=u0,u1
  EngEoNOx Table3 : Lookup_n-D  BreakpointsForDimension1=MAP_FUELCMD  BreakpointsForDimension2=MAP_SPD  Table=MAP_EoNOx  ExtrapMethod=Clip  InternalRulePriority=Speed  RndMeth=Simplest
      settings: InputPortMap=u0,u1
  EngEoPM Table1 : Lookup_n-D  BreakpointsForDimension1=MAP_FUELCMD  BreakpointsForDimension2=MAP_SPD  Table=MAP_EoPM  ExtrapMethod=Clip  InternalRulePriority=Speed  RndMeth=Simplest
      settings: InputPortMap=u0,u1
  EngFuel Table : Lookup_n-D  BreakpointsForDimension1=MAP_FUELCMD  BreakpointsForDimension2=MAP_SPD  Table=MAP_FUEL  ExtrapMethod=Clip  InternalRulePriority=Speed  RndMeth=Simplest
      settings: InputPortMap=u0,u1
  EngPwr Table : Lookup_n-D  BreakpointsForDimension1=MAP_FUELCMD  BreakpointsForDimension2=MAP_SPD  Table=MAP_POWER  ExtrapMethod=Clip  InternalRulePriority=Speed  RndMeth=Simplest
      settings: InputPortMap=u0,u1
  EngSpd2EngTrq1 : Subsystem  Commented=on
  EngSpd2EngTrq2 : Subsystem
  EngTemp Table : Lookup_n-D  BreakpointsForDimension1=MAP_FUELCMD  BreakpointsForDimension2=MAP_SPD  Table=MAP_TEMPERATURE  ExtrapMethod=Clip  InternalRulePriority=Speed  RndMeth=Simplest
      settings: InputPortMap=u0,u1
  Gain{,2..7} (7 alike) : Gain  Gain=1000
  Gain1 : Gain  Gain=0.001
  Gain8 : Gain  Gain=1/3.6
  Gain9 : Gain  Gain=3.6
  Idle : Constant  Value=IdleThrottle
  L/(kW*h) : Lookup_n-D  NumberOfTableDimensions=1  BreakpointsForDimension1=EngSpd  Table=EngCsup  InternalRulePriority=Speed  RndMeth=Simplest
  Manual Switch : ManualSwitch
  Manual Switch1 : ManualSwitch
  Product : Product
  Product1 : Product
  Pulse Generator : DiscretePulseGenerator  PulseType=Time based  Period=0.01  PulseWidth=50
  Rate Limiter : RateLimiter  FallingSlewLimit=-10  SampleTimeMode=inherited
  Scope : Scope  NumInputPorts=4
  Scope1 : Scope
  Switch : Switch  Criteria=u2 > Threshold  SaturateOnIntegerOverflow=off  InputSameDT=off
  rpm2rad/s : Gain  Gain=1/9.55
  EngTrq [Nm] : Outport
  EngInfo : Outport  Port=2
  wires:
  Gain8/1 -> Manual Switch/1  "EngFuel[mL/s]"
  Rate Limiter/1 -> EngSpd2EngTrq2/2(throttle)
  Gain2/1 -> Manual Switch/2
  Gain/1 -> Gain9/1, Bus Creator/4  "EngAir[g/s]"
  EngEoCO2 Table4/1 -> Gain6/1
  EngAir Table/1 -> Gain/1
  EngPwr Table/1 -> Manual Switch1/2
  [FUELCMD] -> EngEEoCO Table2/1
  [FUELCMD] -> EngEoPM Table1/1
  [SPD] -> EngPwr Table/2
  Manual Switch1/1 -> Bus Creator/2  "EngPwr[kW]"
  EngFuel Table/1 -> Gain2/1
  [SPD] -> EngAir Table/2
  EngSpd [rpm]/1 -> Scope/1, EngSpd2EngTrq2/1(speed), [SPD], L/(kW*h)/1, rpm2rad/s/1  "EngSpd[rpm]"
  EngTemp Table/1 -> Display1/1, Bus Creator/5  "EngTemp[K]"
  Gain3/1 -> Display3/1, Bus Creator/7  "EngEoHC[g/s]"
  EngEEoCO Table2/1 -> Gain4/1
  EngSpd2EngTrq2/1(Torque) -> Scope/4, Bus Creator/1, EngTrq [Nm]/1, Scope/2, Product/1  "EngTrq[Nm]"
  EngEoPM Table1/1 -> Gain7/1
  EngEoNOx Table3/1 -> Gain5/1
  LiftCmd [-]/1 -> Switch/2
  [SPD] -> EngEoNOx Table3/2
  [FUELCMD] -> EngEoNOx Table3/1
  Gain4/1 -> Display4/1, Bus Creator/8  "EngEEoCO[g/s]"
  EngEff Table/1 -> Display2/1, Bus Creator/6  "EngEff[g/kwh]"
  Gain6/1 -> Display6/1, Bus Creator/10  "EngEoCO2[g/s]"
  [FUELCMD] -> EngEoHC Table1/1
  Gain5/1 -> Display5/1, Bus Creator/9  "EngEoNOx[g/s]"
  [SPD] -> EngEoCO2 Table4/2
  EngEoHC Table1/1 -> Gain3/1
  [FUELCMD] -> EngTemp Table/1
  [FUELCMD] -> EngEff Table/1
  [SPD] -> EngEEoCO Table2/2
  [FUELCMD] -> EngFuel Table/1
  [FUELCMD] -> EngAir Table/1
  [SPD] -> EngEff Table/2
  rpm2rad/s/1 -> Product/2
  Bus Creator/1 -> EngInfo/1
  Product1/1 -> Gain8/1  "FuelRate[L/h]"
  Product/1 -> Gain1/1
  [FUELCMD] -> EngEoCO2 Table4/1
  Idle/1 -> Switch/1
  Manual Switch/1 -> Bus Creator/3  "EngFuel[mL/s]"
  [SPD] -> EngTemp Table/2
  [SPD] -> EngEoHC Table1/2
  [FUELCMD] -> EngPwr Table/1
  Switch/1 -> Rate Limiter/1
  L/(kW*h)/1 -> Product1/2
  [SPD] -> EngFuel Table/2
  Gain1/1 -> Manual Switch1/1, Scope/3, Product1/1  "EngPwr[kW]"
  ThrottleCmd [-]/1 -> [FUELCMD], Switch/3
  [SPD] -> EngEoPM Table1/2
  Gain7/1 -> Bus Creator/11, Display7/1  "EngEoPM[g/s]"
  Gain9/1 -> Scope1/1  "EngAirIntake[kg/h]"
  Pulse Generator/1 -> EngSpd2EngTrq2/Trigger

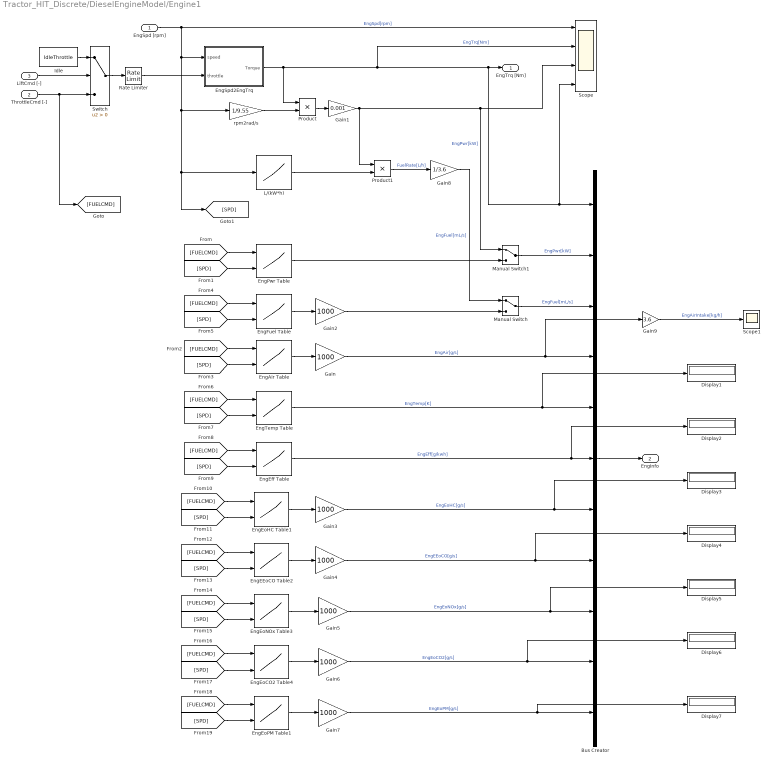
== system Tractor_HIT_Discrete/DieselEngineModel/Engine1 ==
  EngSpd [rpm] : Inport
  ThrottleCmd [-] : Inport  Port=2
  LiftCmd [-] : Inport  Port=3
  Bus Creator : BusCreator  Inputs=11
  Display{1..7} (7 alike) : Display
  EngAir Table : Lookup_n-D  BreakpointsForDimension1=MAP_FUELCMD  BreakpointsForDimension2=MAP_SPD  Table=MAP_AIR  ExtrapMethod=Clip  InternalRulePriority=Speed  RndMeth=Simplest
      settings: InputPortMap=u0,u1
  EngEEoCO Table2 : Lookup_n-D  BreakpointsForDimension1=MAP_FUELCMD  BreakpointsForDimension2=MAP_SPD  Table=MAP_EoCO  ExtrapMethod=Clip  InternalRulePriority=Speed  RndMeth=Simplest
      settings: InputPortMap=u0,u1
  EngEff Table : Lookup_n-D  BreakpointsForDimension1=MAP_FUELCMD  BreakpointsForDimension2=MAP_SPD  Table=MAP_EFF  ExtrapMethod=Clip  InternalRulePriority=Speed  RndMeth=Simplest
      settings: InputPortMap=u0,u1
  EngEoCO2 Table4 : Lookup_n-D  BreakpointsForDimension1=MAP_FUELCMD  BreakpointsForDimension2=MAP_SPD  Table=MAP_EoCO2  ExtrapMethod=Clip  InternalRulePriority=Speed  RndMeth=Simplest
      settings: InputPortMap=u0,u1
  EngEoHC Table1 : Lookup_n-D  BreakpointsForDimension1=MAP_FUELCMD  BreakpointsForDimension2=MAP_SPD  Table=MAP_EoHC  ExtrapMethod=Clip  InternalRulePriority=Speed  RndMeth=Simplest
      settings: InputPortMap=u0,u1
  EngEoNOx Table3 : Lookup_n-D  BreakpointsForDimension1=MAP_FUELCMD  BreakpointsForDimension2=MAP_SPD  Table=MAP_EoNOx  ExtrapMethod=Clip  InternalRulePriority=Speed  RndMeth=Simplest
      settings: InputPortMap=u0,u1
  EngEoPM Table1 : Lookup_n-D  BreakpointsForDimension1=MAP_FUELCMD  BreakpointsForDimension2=MAP_SPD  Table=MAP_EoPM  ExtrapMethod=Clip  InternalRulePriority=Speed  RndMeth=Simplest
      settings: InputPortMap=u0,u1
  EngFuel Table : Lookup_n-D  BreakpointsForDimension1=MAP_FUELCMD  BreakpointsForDimension2=MAP_SPD  Table=MAP_FUEL  ExtrapMethod=Clip  InternalRulePriority=Speed  RndMeth=Simplest
      settings: InputPortMap=u0,u1
  EngPwr Table : Lookup_n-D  BreakpointsForDimension1=MAP_FUELCMD  BreakpointsForDimension2=MAP_SPD  Table=MAP_POWER  ExtrapMethod=Clip  InternalRulePriority=Speed  RndMeth=Simplest
      settings: InputPortMap=u0,u1
  EngSpd2EngTrq : Subsystem
  EngTemp Table : Lookup_n-D  BreakpointsForDimension1=MAP_FUELCMD  BreakpointsForDimension2=MAP_SPD  Table=MAP_TEMPERATURE  ExtrapMethod=Clip  InternalRulePriority=Speed  RndMeth=Simplest
      settings: InputPortMap=u0,u1
  Gain{,2..7} (7 alike) : Gain  Gain=1000
  Gain1 : Gain  Gain=0.001
  Gain8 : Gain  Gain=1/3.6
  Gain9 : Gain  Gain=3.6
  Idle : Constant  Value=IdleThrottle
  L/(kW*h) : Lookup_n-D  NumberOfTableDimensions=1  BreakpointsForDimension1=EngSpd  Table=EngCsup  InternalRulePriority=Speed  RndMeth=Simplest
  Manual Switch : ManualSwitch
  Manual Switch1 : ManualSwitch
  Product : Product
  Product1 : Product
  Rate Limiter : RateLimiter  FallingSlewLimit=-10  SampleTimeMode=inherited
  Scope : Scope  NumInputPorts=4
  Scope1 : Scope
  Switch : Switch  Criteria=u2 > Threshold  SaturateOnIntegerOverflow=off  InputSameDT=off
  rpm2rad/s : Gain  Gain=1/9.55
  EngTrq [Nm] : Outport
  EngInfo : Outport  Port=2
  wires:
  Gain9/1 -> Scope1/1  "EngAirIntake[kg/h]"
  Gain7/1 -> Display7/1, Bus Creator/11  "EngEoPM[g/s]"
  [SPD] -> EngEoPM Table1/2
  ThrottleCmd [-]/1 -> Switch/3, [FUELCMD]
  Gain1/1 -> Product1/1, Scope/3, Manual Switch1/1  "EngPwr[kW]"
  [SPD] -> EngFuel Table/2
  L/(kW*h)/1 -> Product1/2
  Switch/1 -> Rate Limiter/1
  [FUELCMD] -> EngPwr Table/1
  [SPD] -> EngEoHC Table1/2
  [SPD] -> EngTemp Table/2
  Manual Switch/1 -> Bus Creator/3  "EngFuel[mL/s]"
  Idle/1 -> Switch/1
  [FUELCMD] -> EngEoCO2 Table4/1
  Product/1 -> Gain1/1
  Product1/1 -> Gain8/1  "FuelRate[L/h]"
  Bus Creator/1 -> EngInfo/1
  rpm2rad/s/1 -> Product/2
  [SPD] -> EngEff Table/2
  [FUELCMD] -> EngAir Table/1
  [FUELCMD] -> EngFuel Table/1
  [SPD] -> EngEEoCO Table2/2
  [FUELCMD] -> EngEff Table/1
  [FUELCMD] -> EngTemp Table/1
  EngEoHC Table1/1 -> Gain3/1
  [SPD] -> EngEoCO2 Table4/2
  Gain5/1 -> Bus Creator/9, Display5/1  "EngEoNOx[g/s]"
  [FUELCMD] -> EngEoHC Table1/1
  Gain6/1 -> Bus Creator/10, Display6/1  "EngEoCO2[g/s]"
  EngEff Table/1 -> Bus Creator/6, Display2/1  "EngEff[g/kwh]"
  Gain4/1 -> Bus Creator/8, Display4/1  "EngEEoCO[g/s]"
  [FUELCMD] -> EngEoNOx Table3/1
  [SPD] -> EngEoNOx Table3/2
  LiftCmd [-]/1 -> Switch/2
  EngEoNOx Table3/1 -> Gain5/1
  EngEoPM Table1/1 -> Gain7/1
  EngSpd2EngTrq/1(Torque) -> Product/1, Scope/2, EngTrq [Nm]/1, Bus Creator/1, Scope/4  "EngTrq[Nm]"
  EngEEoCO Table2/1 -> Gain4/1
  Gain3/1 -> Bus Creator/7, Display3/1  "EngEoHC[g/s]"
  EngTemp Table/1 -> Bus Creator/5, Display1/1  "EngTemp[K]"
  EngSpd [rpm]/1 -> rpm2rad/s/1, L/(kW*h)/1, [SPD], EngSpd2EngTrq/1(speed), Scope/1  "EngSpd[rpm]"
  [SPD] -> EngAir Table/2
  EngFuel Table/1 -> Gain2/1
  Manual Switch1/1 -> Bus Creator/2  "EngPwr[kW]"
  [SPD] -> EngPwr Table/2
  [FUELCMD] -> EngEoPM Table1/1
  [FUELCMD] -> EngEEoCO Table2/1
  EngPwr Table/1 -> Manual Switch1/2
  EngAir Table/1 -> Gain/1
  EngEoCO2 Table4/1 -> Gain6/1
  Gain/1 -> Bus Creator/4, Gain9/1  "EngAir[g/s]"
  Gain2/1 -> Manual Switch/2
  Rate Limiter/1 -> EngSpd2EngTrq/2(throttle)
  Gain8/1 -> Manual Switch/1  "EngFuel[mL/s]"

== system Tractor_HIT_Discrete/ECU/ECU ==
  EngineSpd_rpm : Inport
  FuleCyle_mg : Inport  Port=2
  EGRRatio : Inport  Port=3
  RailPrs_kpa : Inport  Port=4
  IntakeMass : Inport  Port=5
  ExhTemp_DOC_in : Inport  Port=6
  ExhTemp_DOC_out : Inport  Port=7
  ExhTemp_DPF_out : Inport  Port=8
  ExhTemp_SCR_out : Inport  Port=9
  ExhMassFlow : Inport  Port=10
  mNOx_SCR_in : Inport  Port=11
  mNOx_SCR_out : Inport  Port=12
  DPF_SootLoad : Inport  Port=13
  DPF_DP : Inport  Port=14
  NH3_Store : Inport  Port=15
  O2_frac : Inport  Port=16
  ThrottleCmd_pct : Inport  Port=17
  ANR : Subsystem
  DPF_REGEN : Subsystem
  EGRCtrl : Subsystem
  SpdCtrl : Subsystem
  Terminator{2..4,6..7} (5 alike) : Terminator
  EngineSpdTgt_rpm : Outport
  FuelCyleTgt_mg : Outport  Port=2
  EGROpeningTgt_pct : Outport  Port=3
  PostInj_Request : Outport  Port=4
  DPF_regen_req : Outport  Port=5
  mUREA_target : Outport  Port=6
  wires:
  SpdCtrl/1(FuelCycle_mg) -> FuelCyleTgt_mg/1
  EngineSpd_rpm/1 -> [EngineSpd_rpm], SpdCtrl/2(EngineSpd_rpm)
  FuleCyle_mg/1 -> EGRCtrl/2(FuleCycle_mg)
  EGRCtrl/1(EGROpeningTgt_pct) -> EGROpeningTgt_pct/1
  EGRRatio/1 -> EGRCtrl/3(EGRRatio)
  RailPrs_kpa/1 -> SpdCtrl/3(RailPrs_kpa)
  IntakeMass/1 -> SpdCtrl/4(IntakeMass)
  [EngineSpd_rpm] -> EGRCtrl/1(EngineSpd_rpm)
  mNOx_SCR_in/1 -> ANR/2(mNOx_SCR_kg/h)
  ANR/1(mUREA_target) -> mUREA_target/1
  ExhTemp_DPF_out/1 -> DPF_REGEN/2(ExhTemp_DPF_out), ANR/1(ExhTemp_DPF_out)
  DPF_SootLoad/1 -> DPF_REGEN/3(DPF_SootLoad)
  ExhMassFlow/1 -> DPF_REGEN/4(ExhMassFlow)
  DPF_REGEN/1(DPF_regen_req) -> DPF_regen_req/1
  ExhTemp_DOC_in/1 -> Terminator4/1
  mNOx_SCR_out/1 -> Terminator2/1
  ExhTemp_SCR_out/1 -> Terminator3/1
  NH3_Store/1 -> Terminator7/1
  O2_frac/1 -> Terminator6/1
  DPF_DP/1 -> DPF_REGEN/5(DPF_DP)
  ExhTemp_DOC_out/1 -> DPF_REGEN/1(ExhTemp_DOC_out)
  [EngineSpd_rpm] -> DPF_REGEN/6(EngineSpd_rpm)
  DPF_REGEN/2(PostInj_Request) -> PostInj_Request/1
  ThrottleCmd_pct/1 -> SpdCtrl/1(ThrottleCmd_pct)
  SpdCtrl/2(EngineSpdTgt_rpm) -> EngineSpdTgt_rpm/1

== system Tractor_HIT_Discrete/Engine/ECU ==
  EngineSpd_rpm : Inport
  FuleCyle_mg : Inport  Port=2
  EGRRatio : Inport  Port=3
  RailPrs_kpa : Inport  Port=4
  IntakeMass : Inport  Port=5
  ExhTemp_DOC_in : Inport  Port=6
  ExhTemp_DOC_out : Inport  Port=7
  ExhTemp_DPF_out : Inport  Port=8
  ExhTemp_SCR_out : Inport  Port=9
  ExhMassFlow : Inport  Port=10
  mNOx_SCR_in : Inport  Port=11
  mNOx_SCR_out : Inport  Port=12
  DPF_SootLoad : Inport  Port=13
  DPF_DP : Inport  Port=14
  NH3_Store : Inport  Port=15
  O2_frac : Inport  Port=16
  ThrottleCmd [-] : Inport  Port=17
  ANR : Subsystem
  DPF_REGEN : Subsystem
  EGRCtrl : Subsystem
  SpdCtrl : Subsystem
  Terminator{2..4,6..7} (5 alike) : Terminator
  EngineSpdTgt_rpm : Outport
  FuelCyleTgt_mg : Outport  Port=2
  EGROpeningTgt_pct : Outport  Port=3
  PostInj_Request : Outport  Port=4
  DPF_regen_req : Outport  Port=5
  mUREA_target : Outport  Port=6
  wires:
  SpdCtrl/1(FuelCycle_mg) -> FuelCyleTgt_mg/1
  EngineSpd_rpm/1 -> [EngineSpd_rpm], SpdCtrl/2(EngineSpd_rpm)
  FuleCyle_mg/1 -> EGRCtrl/2(FuleCycle_mg)
  EGRCtrl/1(EGROpeningTgt_pct) -> EGROpeningTgt_pct/1
  EGRRatio/1 -> EGRCtrl/3(EGRRatio)
  RailPrs_kpa/1 -> SpdCtrl/3(RailPrs_kpa)
  IntakeMass/1 -> SpdCtrl/4(IntakeMass)
  [EngineSpd_rpm] -> EGRCtrl/1(EngineSpd_rpm)
  mNOx_SCR_in/1 -> ANR/2(mNOx_SCR_kg/h)
  ANR/1(mUREA_target) -> mUREA_target/1
  ExhTemp_DPF_out/1 -> DPF_REGEN/2(ExhTemp_DPF_out), ANR/1(ExhTemp_DPF_out)
  DPF_SootLoad/1 -> DPF_REGEN/3(DPF_SootLoad)
  ExhMassFlow/1 -> DPF_REGEN/4(ExhMassFlow)
  DPF_REGEN/1(DPF_regen_req) -> DPF_regen_req/1
  ExhTemp_DOC_in/1 -> Terminator4/1
  mNOx_SCR_out/1 -> Terminator2/1
  ExhTemp_SCR_out/1 -> Terminator3/1
  NH3_Store/1 -> Terminator7/1
  O2_frac/1 -> Terminator6/1
  DPF_DP/1 -> DPF_REGEN/5(DPF_DP)
  ExhTemp_DOC_out/1 -> DPF_REGEN/1(ExhTemp_DOC_out)
  [EngineSpd_rpm] -> DPF_REGEN/6(EngineSpd_rpm)
  DPF_REGEN/2(PostInj_Request) -> PostInj_Request/1
  ThrottleCmd [-]/1 -> SpdCtrl/1(ThrottleCmd [-])
  SpdCtrl/2(EngineSpdTgt_rpm) -> EngineSpdTgt_rpm/1

== system Tractor_HIT_Discrete/Engine/Engine ==
  EngineSpd_rpm : Inport
  FuelCyleTgt_mg : Inport  Port=2
  EGROpeningTgt_pct : Inport  Port=3
  PostInj_Request : Inport  Port=4
  DPF_regen_req : Inport  Port=5
  mUREA_target : Inport  Port=6
  AftertreatmentModel : Subsystem
      settings: PortSchema="{\"entries\":[{\"content\":{\"sides\":[{\"content\":{\"connectorIds\":[\"In1\",\"In2\",\"In3\",\"In4\",\"In5\",\"In6\",\"In7\",\"In8\"]},\"type\":\"ConnectorPlacement.EquallySpacedRectSide\",\"uuid\":\"dc3885dc-d75a-4863-96d4-1450d2f18eb5\"},{\"content\":{\"connectorIds\":[\"Out1\",\"Out2\",\"Out3\",\"Out4\",\"Out5\",\"Out6\",\"Out7\",\"Out8\",\"Out9\",\"Out10\",\"Out11\"],\"side\":\"RIGHT\"},\"type\":\"ConnectorPlacement.EquallySpacedRectSide\",\"uuid\":\"a23f18c1-a3dc-4e15-8495-9e7ba08b1330\"},{\"content\":{\"connectorIds\":[\"In9\",\"In10\"],\"side\":\"TOP\"},\"type\":\"ConnectorPlacement.EquallySpacedRectSide\",\"uuid\":\"68c9c1a9-0c9f-492c-9136-64aa2da3a2c4\"}]},\"type\":\"ConnectorPlacement.EquallySpacedConnector\",\"uuid\":\"43fc83f2-b125-4818-97d9-f8d537b373ba\"}],\"packageUris\":[\"http://schema.mathworks.com/mf0/Connector/R2020b\"],\"version\":\"1.0\"}"
  Terminator : Terminator
  Terminator1 : Terminator
  ThermalModel : Subsystem
      settings: PortSchema="{\"entries\":[{\"content\":{\"sides\":[{\"content\":{\"connectorIds\":[\"In1\"]},\"type\":\"ConnectorPlacement.EquallySpacedRectSide\",\"uuid\":\"cb969e7d-00a7-424a-8652-d2f01214e72a\"},{\"content\":{\"connectorIds\":[\"Out1\",\"Out2\",\"Out3\",\"Out4\",\"Out5\",\"Out6\",\"Out7\",\"Out8\",\"Out9\",\"Out10\",\"Out11\",\"Out12\",\"Out13\",\"Out14\",\"Out15\"],\"side\":\"RIGHT\"},\"type\":\"ConnectorPlacement.EquallySpacedRectSide\",\"uuid\":\"e1483eb6-feba-4067-87e9-6babff0aabb4\"},{\"content\":{\"connectorIds\":[\"In2\",\"In3\",\"In4\"],\"side\":\"TOP\"},\"type\":\"ConnectorPlacement.EquallySpacedRectSide\",\"uuid\":\"cfcf3803-6a1f-4377-9343-ab5e07509018\"},{\"content\":{\"side\":\"BOTTOM\"},\"type\":\"ConnectorPlacement.EquallySpacedRectSide\",\"uuid\":\"7ac90eca-8fa8-4aaf-a947-ddd22b296071\"}]},\"type\":\"ConnectorPlacement.EquallySpacedConnector\",\"uuid\":\"45480179-d528-400e-8737-4cf305bd92e4\"}],\"packageUris\":[\"http://schema.mathworks.com/mf0/Connector/R2020b\"],\"version\":\"1.0\"}"
  EngineTrq_Nm : Outport
  FuelCyle_g : Outport  Port=2
  EGRRatio : Outport  Port=3
  RailPrs_kpa : Outport  Port=4
  IntakeMass_kg/h : Outport  Port=5
  ExhTemp_DOC_in : Outport  Port=6
  ExhTemp_DOC_out : Outport  Port=7
  ExhTemp_DPF_out : Outport  Port=8
  ExhTemp_SCR_out : Outport  Port=9
  ExhMassFlow : Outport  Port=10
  mNOx_SCR_in : Outport  Port=11
  mNOx_SCR_out : Outport  Port=12
  Soot_Load : Outport  Port=13
  DPF_DP : Outport  Port=14
  NH3_Store : Outport  Port=15
  O2_frac : Outport  Port=16
  wires:
  FuelCyleTgt_mg/1 -> ThermalModel/4(FuelCyleTgt_mg)
  EGROpeningTgt_pct/1 -> ThermalModel/3(EGROpeningTgt_pct)
  ThermalModel/3(RailPrs_kpa) -> RailPrs_kpa/1
  ThermalModel/1(FuelCycle_mg) -> FuelCyle_g/1
  ThermalModel/2(EGRRatio) -> EGRRatio/1
  ThermalModel/5(IntakePrs_kpa) -> Terminator1/1
  ThermalModel/6(EngineTrq_Nm) -> EngineTrq_Nm/1
  ThermalModel/9(EGT_c) -> AftertreatmentModel/2(EGT_c)
  ThermalModel/8(ExhMassFlow_kg/h) -> AftertreatmentModel/1(ExhMassFlow_kg/h)
  ThermalModel/11(O2_pct) -> AftertreatmentModel/4(O2_pct)
  ThermalModel/15(PM_kg/h) -> AftertreatmentModel/8(PM_kg/h)
  ThermalModel/13(HC_kg/h) -> AftertreatmentModel/6(HC_kg/h)
  ThermalModel/14(CO_kg/h) -> AftertreatmentModel/7(CO_kg/h)
  ThermalModel/10(ExhPrs_kpa) -> AftertreatmentModel/3(ExhPrs_kpa)
  ThermalModel/12(NOx_kg/h) -> AftertreatmentModel/5(NOx_kg/h)
  ThermalModel/4(IntakeMass_kg/h) -> IntakeMass_kg/h/1
  DPF_regen_req/1 -> AftertreatmentModel/10(DPF_regen_req)
  AftertreatmentModel/1(ExhTemp_DOC_in) -> ExhTemp_DOC_in/1
  AftertreatmentModel/2(ExhTemp_DOC_out) -> ExhTemp_DOC_out/1
  AftertreatmentModel/3(ExhTemp_DPF_out) -> ExhTemp_DPF_out/1
  AftertreatmentModel/4(ExhTemp_SCR_out) -> ExhTemp_SCR_out/1
  AftertreatmentModel/5(ExhMassFlow) -> ExhMassFlow/1
  AftertreatmentModel/6(mNOx_SCR_in) -> mNOx_SCR_in/1
  AftertreatmentModel/7(mNOx_SCR_out) -> mNOx_SCR_out/1
  AftertreatmentModel/8(Soot_Load) -> Soot_Load/1
  AftertreatmentModel/9(DPF_DP) -> DPF_DP/1
  AftertreatmentModel/10(NH3_Store) -> NH3_Store/1
  AftertreatmentModel/11(O2_frac) -> O2_frac/1
  mUREA_target/1 -> AftertreatmentModel/9(mUREA_target)
  ThermalModel/7(BSFC_kg/h) -> Terminator/1
  PostInj_Request/1 -> ThermalModel/2(PostInj_Request)
  EngineSpd_rpm/1 -> ThermalModel/1(EngineSpd_rpm)
